simulink library "Damper_Control_Axle2"  (R2025a)
settings: Solver=VariableStepAuto  StartTime=0.0  StopTime=10.0  RelTol=1e-3
libraries: Damper_Control x2, Vehicle_Outputs x1
Description:
  | Copyright 2026 The MathWorks, Inc.
settings Model: Creator=smiller  LastModifiedBy=smiller
settings OptimizationCC: ReuseModelBlockBuffer=off
settings ModelReferenceCC: EnableRefExpFcnMdlSchedulingChecks=on
settings RTWCC: GPUComputeCapability=3.5

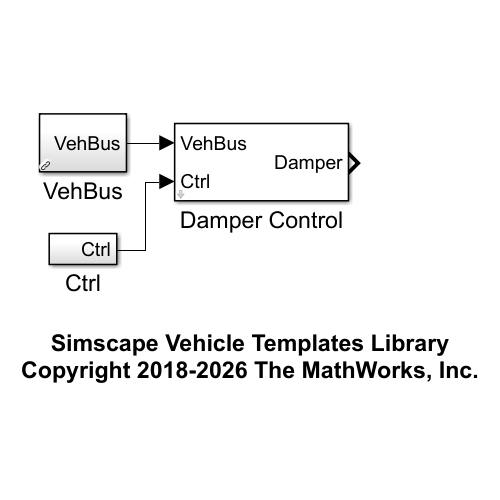
[thumbnail: Simulink's stored preview of the top-level diagram]
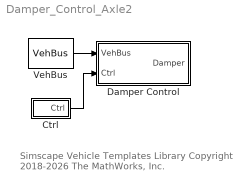
== system Damper_Control_Axle2 ==
  note: Simscape Vehicle Templates Library
      | Copyright 2018-2026 The MathWorks, Inc.
  Ctrl : Subsystem
  Damper Control : Subsystem  mask(Damper Control, Two Axle){popup_damper_control_A1=None, popup_damper_control_A2=None}
      mask prompts: popup_damper_control_A1 "Damper Control Axle 1"; popup_damper_control_A2 "Damper Control Axle 2"
      mask help: Configurable damper control for two axles, left and right sides.
      mask TypeOptions popup_damper_control_A1: Damper Control A1/popup_damper_control
      mask TypeOptions popup_damper_control_A2: Damper Control A2/popup_damper_control
  VehBus : Vehicle_Outputs/VehBus  SystemSampleTime=-1  VariantActivationTime=update diagram  EmptyChoice=off  PassThrough=off  PassThroughVariantControl=(default)  EmptyChoiceVariantControl=(default)  AllowFlexibleInterface=on  Latency=0  AutoFrameSizeCalculation=off
  wires:
  VehBus/1 -> Damper Control/1(VehBus)
  Ctrl/1(Ctrl) -> Damper Control/2(Ctrl)

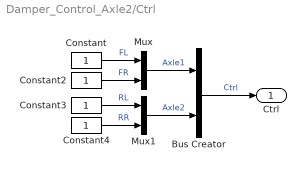
== system Damper_Control_Axle2/Ctrl ==
  Bus Creator : BusCreator  Inputs=2
  Constant{,2..4} (4 alike) : Constant
  Mux : Mux  Inputs=2
  Mux1 : Mux  Inputs=2
  Ctrl : Outport
  wires:
  Mux/1 -> Bus Creator/1  "Axle1"
  Mux1/1 -> Bus Creator/2  "Axle2"
  Bus Creator/1 -> Ctrl/1  "Ctrl"
  Constant/1 -> Mux/1  "FL"
  Constant2/1 -> Mux/2  "FR"
  Constant4/1 -> Mux1/2  "RR"
  Constant3/1 -> Mux1/1  "RL"

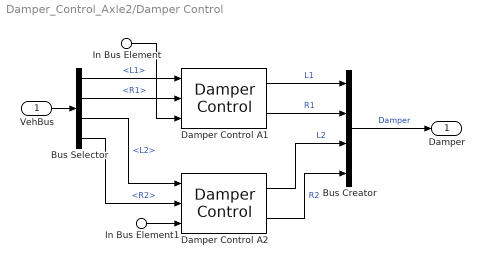
== system Damper_Control_Axle2/Damper Control ==
  VehBus : Inport
  In Bus Element : Inport  Port=2  PortName=Ctrl  Element=Axle1
  In Bus Element1 : Inport  Port=2  PortName=Ctrl  Element=Axle2
  Bus Creator : BusCreator  Inputs=4
  Bus Selector : BusSelector  OutputSignals=Chassis.Damper.L1,Chassis.Damper.R1,Chassis.Damper.L2,Chassis.Damper.R2
  Damper Control A1 : Damper_Control/Damper Control   VariantControl=Choice  LabelModeActiveChoice=None  popup_damper_control=None  ControlDamper=Control.Damper.Axle1
      settings: AttributesFormatString=%<popup_damper_control>
  Damper Control A2 : Damper_Control/Damper Control   VariantControl=Choice  LabelModeActiveChoice=None  popup_damper_control=None  ControlDamper=Control.Damper.Axle2
      settings: AttributesFormatString=%<popup_damper_control>
  Damper : Outport
  wires:
  VehBus/1 -> Bus Selector/1
  Damper Control A1/1 -> Bus Creator/1  "L1"
  Bus Selector/1 -> Damper Control A1/1  "<L1>"
  Bus Selector/2 -> Damper Control A1/2  "<R1>"
  Bus Selector/3 -> Damper Control A2/1  "<L2>"
  Bus Selector/4 -> Damper Control A2/2  "<R2>"
  Bus Creator/1 -> Damper/1  "Damper"
  Damper Control A1/2 -> Bus Creator/2  "R1"
  Damper Control A2/1 -> Bus Creator/3  "L2"
  Damper Control A2/2 -> Bus Creator/4  "R2"
  In Bus Element/1 -> Damper Control A1/3
  In Bus Element1/1 -> Damper Control A2/3
